simulink library "Model_DG_Grid_Following_Converter"  (R2023b)
settings: Solver=VariableStepAuto  StartTime=0.0  StopTime=10.0  RelTol=1e-3
undefined symbols (not defined in the file): K_Matching, Luenberger_Gain, ss_plant, ss_ref, Ts_Matching
settings Model: Creator=winkens  LastModifiedBy=a.och
settings SolverCC: AlgebraicLoopSolver=TrustRegion
settings OptimizationCC: ReuseModelBlockBuffer=off
settings DebuggingCC: UnconnectedInputMsg=warning  UnconnectedOutputMsg=warning  UnconnectedLineMsg=warning
settings ModelReferenceCC: EnableRefExpFcnMdlSchedulingChecks=on
settings RTWCC: DLArmComputeVersion=19.05

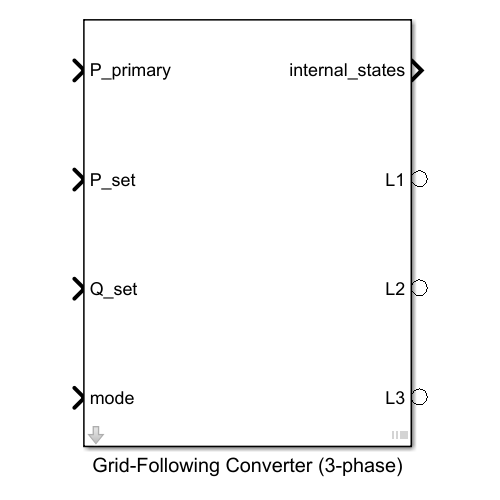
[thumbnail: Simulink's stored preview of the top-level diagram]
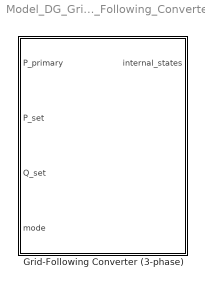
== system Model_DG_Grid_Following_Converter ==
  Grid-Following Converter (3-phase) : Subsystem  mask{S_n=30e3, P_binst=30e3, V_n_phph=400, f_n=50, send_messages=on, T_s_ctrl=1e-4, T_s_PWM_meas=1e-4, T_s_SPS=1e-4, datatype='double', swModeling=Average Model, f_sw=5e3, L_filter_conv_pu=[ 0.0001 0.05097 ], C_filter_pu=[ 0.06875 0.04569 ], L_filter_grid_pu=[ 0.01 0.04 ], withTransformer=Direct grid coupling of converter, V_n_grid_phph=20e3, RL_Trafo_Conv=[ 0.005 0.02 ], RL_Trafo_Grid=[ 0.005 0.02 ], Rm=500, Lm=500, meas_LPF=on, meas_LPF_f_cutoff=2500, prot_variant=tDMSquared warnings only, prot_v_ac_max=1.1, prot_t_ac_max=0.1, prot_v_ac_maxmax=1.25, prot_t_ac_maxmax=0.1, prot_v_ac_min=0.8, prot_t_ac_min=3, prot_v_ac_minmin=0.45, prot_t_ac_minmin=0.3, prot_f_ac_max=51.5, prot_t_f_ac_max=0.1, prot_f_ac_maxmax=52.5, prot_t_f_ac_maxmax=10, prot_f_ac_min=47.5, prot_t_f_ac_min=0.1, prot_i_ac_max=1.3, unitCtrlMode=VDE 4110, VDE4110_Pf_DBlow=49.8, VDE4110_Pf_DBhigh=50.2, VDE4110_Pf_droop=5, VDE4110_Pf_dPdt_max=1, VDE4110_Pf_T_LPF=33e-3, VDE4110_Pf_isStorage=on, ts_matching=0%Ts_Matching, k_matching=0%K_Matching, plant_ref_m=0%ss_ref, plant_model_m=0%ss_plant, luenberger_m=0%Luenberger_Gain, VDE4110_Q_Mode=(a) Q(V)-curve, VDE4110_Q_T_PT1=3.33, VDE4110_uq0ref=1, VDE4110_qmax=0.33, VDE4110_umax=1.04, VDE4110_deadband=0, VDE4110_p_pu=[0.1, 0.5, 0.6, 0.9, 1.0], VDE4110_q_pu=[0.0, 0.0, -0.05, -0.33, -0.33], VDE4110_p1=[0.94, 0.33], VDE4110_p2=[0.96, 0], VDE4110_p3=[1.04, 0], VDE4110_p4=[1.06, -0.33], VDE4110_cosphi_ref=1, VDE4110_Q_direction=Inductive Q injection, InnerCtrl_PQ_Ctrl_Mode=Closed loop, InnerCtrl_Kp_PQ=0.6, InnerCtrl_Ki_PQ=3.2, InnerCtrl_Kp=0.6, InnerCtrl_Ki=0.6, InnerCtrl_v_conv_max=1.3, InnerCtrl_i_conv_max=1.1, InnerCtrl_AD_activated=on, InnerCtrl_AD_Rvirt=0.2}
      mask prompts: S_n "Nominal Apparent Power [VA]"; P_binst "Installed Active Power [W]"; V_n_phph "Nominal Converter Voltage (rms, phase-to-phase) [V]"; f_n "Nominal Frequency [Hz]"; send_messages "Send tDMSquared info messages"; T_s_ctrl "Controller sample time [s]"; T_s_PWM_meas "PWM and measurements sample time [s]"; T_s_SPS "Simscape SPS sample time [s]"; datatype "Signal data type"; swModeling "Model type:"; f_sw "Switching Frequency [Hz]"; L_filter_conv_pu "Impedance of Converter-Side-Inductor [ R L ] (p.u.)"; C_filter_pu "Impedance of Filter Capacitor [ R C ] (p.u.)"; L_filter_grid_pu "Impedance of Grid-Side Inductor* [ R L ] (p.u.)"; V_n_grid_phph "Nominal Grid Voltage (rms, phase-to-phase) [V]"; RL_Trafo_Conv "Converter-Side Impedance [ R L ] (pu)"; RL_Trafo_Grid "Grid-Side Impedance [ R L ] (pu)"; Rm "Magnetization resistance Rm (pu)"; Lm "Magnetization inductance Lm (pu)"; meas_LPF "Apply low pass filtering to measured signals"; meas_LPF_f_cutoff "Cutoff frequency of the low pass filter applied to measurements [Hz]"; prot_variant "Protection variant"; prot_v_ac_max "Maximum AC voltage [% nom. value]"; prot_t_ac_max "Maximum AC voltage timing [s]"; prot_v_ac_maxmax "Upper Maximum AC voltage [% nom. value]"; prot_t_ac_maxmax "Upper Maximum AC voltage timing [s]"; prot_v_ac_min "Upper Minimum AC voltage [% nom. value]"; prot_t_ac_min "Upper Minimum AC voltage timing [s]"; prot_v_ac_minmin "Lower Minimum AC voltage [% nom. value]"; prot_t_ac_minmin "Lower Minimum AC voltage timing [s]"; prot_f_ac_max "Maximum AC frequency [Hz]"; prot_t_f_ac_max "Maximum AC frequency timing [s]"; prot_f_ac_maxmax "Upper Maximum AC frequency [Hz]"; prot_t_f_ac_maxmax "Upper Maximum AC frequency timing [s]"; prot_f_ac_min "Minimum AC frequency [Hz]"; prot_t_f_ac_min "Minimum AC frequency timing [s]"; prot_i_ac_max "Maximum AC current [% nom. value]"; unitCtrlMode "Unit Control Mode"; VDE4110_Pf_DBlow "P(f) Deadband Lower Limit [Hz]"; VDE4110_Pf_DBhigh "P(f) Deadband Upper Limit [Hz]"; VDE4110_Pf_droop "P(f) Droop [(df/f_n)/(dP/Pref)] [%]"; VDE4110_Pf_dPdt_max "P(f) Maximum dP/dt [pu / s]"; VDE4110_Pf_T_LPF "P(f) time constant of active power PT1 delay [s]"; VDE4110_Pf_isStorage "Generation Unit Is Energy Storage"; ts_matching "Time Constant"; k_matching "Feedback Gain"; plant_ref_m "Reference Model"; plant_model_m "Plant Model"; luenberger_m "Luenberger Gain"; VDE4110_Q_Mode "Q-Control Mode"; VDE4110_Q_T_PT1 "Time constant of reactive power PT1 delay [s]"; VDE4110_uq0ref "U_Q0ref [pu]"; VDE4110_qmax "|Q_max| [pu]"; VDE4110_umax "U_max [pu]"; VDE4110_deadband "Voltage Deadband [+- %]"; VDE4110_p_pu "P_grid points [pu]"; VDE4110_q_pu "Q_grid points [pu]"; VDE4110_p1 "P1 [V_grid, Q_grid] [pu]"; VDE4110_p2 "P2 [V_grid, Q_grid] [pu]"; VDE4110_p3 "P3 [V_grid, Q_grid] [pu]"; VDE4110_p4 "P4 [V_grid, Q_grid] [pu]"; VDE4110_cosphi_ref "cos(phi)"; InnerCtrl_PQ_Ctrl_Mode "Control mode"; InnerCtrl_Kp_PQ "Power controller proportional gain [p.u.]"; InnerCtrl_Ki_PQ "Power controller integral gain [p.u.]"; InnerCtrl_Kp "Current Controller Proportional Gain [p.u.]"; InnerCtrl_Ki "Current Controller Integral Gain [p.u.]"; InnerCtrl_v_conv_max "Converter voltage maximum value (limit) [p.u.]"; InnerCtrl_i_conv_max "Converter current maximum value (limit) [p.u.]"; InnerCtrl_AD_activated "Active damping activated"; InnerCtrl_AD_Rvirt "Virtual resistor for active damping (in series with conv.-side inductance) [p.u.]"
      mask init:
      | % Initialize nominal grid voltage
      | if (withTransformer == 1)
      |     V_n_grid_phph = V_n_phph;
      | end
      mask TypeOptions swModeling: Average Model | Ideal Switches
      mask TypeOptions withTransformer: Direct grid coupling of converter | Grid coupling using transformer
      mask Callback withTransformer:
      | msk = Simulink.Mask.get(gcb);
      | p = msk.Parameters;
      | if strcmp(get_param(gcb, 'withTransformer'), 'Grid coupling using transformer')
      |     %with Transformer
      |     p(16).Visible = 'on';
      |     p(17).Visible = 'on';
      |     p(18).Visible = 'on';
      |     p(19).Visible = 'on';
      |     p(20).Visible = 'on';
      | else
      |     %without Transformer
      |     p(16).Visible = 'off';
      |     p(17).Visible = 'off';
      |     p(18).Visible = 'off';
      |     p(19).Visible = 'off';
      |     p(20).Visible = 'off';
      | end
      mask TypeOptions prot_variant: Hardware protection | tDMSquared warnings only | deactivated | VDE AR
      mask Callback prot_variant:
      | msk = Simulink.Mask.get(gcb);
      | if strcmp(get_param(gcb, 'prot_variant'), 'VDE AR')
      |     msk.getParameter('prot_v_ac_max').Visible ='on';
      |     msk.getParameter('prot_i_ac_max').Visible ='on';
      |     msk.getParameter('prot_t_ac_max').Visible = 'on';
      |     msk.getParameter('prot_v_ac_maxmax').Visible = 'on';
      |     msk.getParameter('prot_t_ac_maxmax').Visible = 'on';
      |     msk.getParameter('prot_v_ac_min').Visible = 'on';
      |     msk.getParameter('prot_t_ac_min').Visible = 'on';
      |     msk.getParameter('prot_v_ac_minmin').Visible = 'on';
      |     msk.getParameter('prot_t_ac_minmin').Visible = 'on';
      |     msk.getParameter('prot_f_ac_max').Visible = 'on';
      |     msk.getParameter('prot_t_f_ac_max').Visible = 'on';
      |     msk.getParameter('prot_f_ac_maxmax').Visible = 'on';
      |     msk.getParameter('prot_t_f_ac_maxmax').Visible = 'on';
      |     msk.getParameter('prot_f_ac_min').Visible = 'on';
      |     msk.getParameter('prot_t_f_ac_min').Visible = 'on';
      | elseif strcmp(get_param(gcb, 'prot_variant'), 'deactivated')
      |     msk.getParameter('prot_v_ac_max').Visible ='off';
      |     msk.getParameter('prot_i_ac_max').Visible ='off';
      |     msk.getParameter('prot_t_ac_max').Visible = 'off';
      |     msk.getParameter('prot_v_ac_maxmax').Visible = 'off';
      |     msk.getParameter('prot_t_ac_maxmax').Visible = 'off';
      |     msk.getParameter('prot_v_ac_min').Visible = 'off';
      |     msk.getParameter('prot_t_ac_min').Visible = 'off';
      |     msk.getParameter('prot_v_ac_minmin').Visible = 'off';
      |     msk.getParameter('prot_t_ac_minmin').Visible = 'off';
      |     msk.getParameter('prot_f_ac_max').Visible = 'off';
      |     msk.getParameter('prot_t_f_ac_max').Visible = 'off';
      |     msk.getParameter('prot_f_ac_maxmax').Visible = 'off';
      |     msk.getParameter('prot_t_f_ac_maxmax').Visible = 'off';
      |     msk.getParameter('prot_f_ac_min').Visible = 'off';
      |     msk.getParameter('prot_t_f_ac_min').Visible = 'off';
      | else
      |     msk.getParameter('prot_v_ac_max').Visible ='on';
      |     msk.getParameter('prot_i_ac_max').Visible ='on';
      |     msk.getParameter('prot_t_ac_max').Visible = 'off';
      |     msk.getParameter('prot_v_ac_maxmax').Visible = 'off';
      |     msk.getParameter('prot_t_ac_maxmax').Visible = 'off';
      |     msk.getParameter('prot_v_ac_min').Visible = 'off';
      |     msk.getParameter('prot_t_ac_min').Visible = 'off';
      |     msk.getParameter('prot_v_ac_minmin').Visible = 'off';
      |     msk.getParameter('prot_t_ac_minmin').Visible = 'off';
      |     msk.getParameter('prot_f_ac_max').Visible = 'off';
      |     msk.getParameter('prot_t_f_ac_max').Visible = 'off';
      |     msk.getParameter('prot_f_ac_maxmax').Visible = 'off';
      |     msk.getParameter('prot_t_f_ac_maxmax').Visible = 'off';
      |     msk.getParameter('prot_f_ac_min').Visible = 'off';
      |     msk.getParameter('prot_t_f_ac_min').Visible = 'off';
      | end
      mask TypeOptions unitCtrlMode: VDE 4110 | Matching Control | No Unit Control
      mask Callback unitCtrlMode:
      | toggleComment = @(s) regexprep( ...
      |     regexprep(s,'^$','0'), ...       % leere Eingabe → '0'
      |     '^(?!0%)(.*)', ...               % Negative Lookahead: wenn nicht '0%' am Anfang
      |     '0%$1' ...                       % dann '0%' voranstellen
      | );
      | 
      | removeComment = @(s) regexprep( ...
      |     regexprep(s,'^$','0'), ...       % leere Eingabe → '0'
      |     '^0%', ...                       % wenn '0%' am Anfang steht
      |     '' ...                           % entferne es
      | );
      |     m = Simulink.Mask.get(gcb);
      | 
      |     modeStr = get_param(gcb, 'unitCtrlMode');
      | 
      |     % 3) Liste der zu „auskommentierenden“ Controls je Modus
      |     vdeControls      = {'VDE4110_Pf_dPdt_max', 'VDE4110_Pf_DBlow', 'VDE4110_Pf_DBhigh', 'VDE4110_Pf_droop', 'VDE4110_Pf_T_LPF'};
      |     matchingControls = {'ts_matching', 'k_matching', 'plant_ref_m', 'plant_model_m', 'luenberger_m'};
      | 
      |     switch modeStr
      |         case 'VDE 4110'
      |             m.getDialogControl('paramboxVDE4110').Visible = 'on';
      |             m.getDialogControl('paramboxMatching').Visible = 'off';
      |             m.getDialogControl('paramboxReactiveCtrl').Visible = 'on';
      |             % → Matching-Felder a u s k o m m e n t i e r e n
      |             for i = 1:numel(matchingControls)
      |                 set_param(gcb, matchingControls{i}, (toggleComment(get_param(gcb, matchingControls{i}))));
      |             end
      |             % → VDE-Felder e n t k o m m e n t i e r e n
      |             for i = 1:numel(vdeControls)
      |                 set_param(gcb, vdeControls{i}, (removeComment(get_param(gcb, vdeControls{i}))));
      |             end
      | 
      |         case 'Matching Control'
      |             m.getDialogControl('paramboxVDE4110').Visible = 'off';
      |             m.getDialogControl('paramboxMatching').Visible = 'on';
      |             m.getDialogControl('paramboxReactiveCtrl').Visible = 'on';
      |             % → VDE-Felder a u s k o m m e n t i e r e n
      |             for i = 1:numel(vdeControls)
      |                 set_param(gcb, vdeControls{i}, (toggleComment(get_param(gcb, vdeControls{i}))));
      |             end
      |             % → Matching-Felder e n t k o m m e n t i e r e n
      |             for i = 1:numel(matchingControls)
      |                 set_param(gcb, matchingControls{i}, (removeComment(get_param(gcb, matchingControls{i}))));
      |             end
      |         case 'No Unit Control'
      |             m.getDialogControl('paramboxVDE4110').Visible = 'off';
      |             m.getDialogControl('paramboxMatching').Visible = 'off';
      |             m.getDialogControl('paramboxReactiveCtrl').Visible = 'off';
      |             % → VDE-Felder a u s k o m m e n t i e r e n
      |             for i = 1:numel(vdeControls)
      |                 set_param(gcb, vdeControls{i}, (toggleComment(get_param(gcb, vdeControls{i}))));
      |             end
      |             % → Matching-Felder e n t k o m m e n t i e r e n
      |             for i = 1:numel(matchingControls)
      |                 set_param(gcb, matchingControls{i}, (toggleComment(get_param(gcb, matchingControls{i}))));
      |             end
      |     end
      mask TypeOptions VDE4110_Q_Mode: (a) Q(V)-curve | (b) Q(P)-curve | (c) Constant Q with Q(V)-limitation | (d) Constant cos(phi)
      mask Callback VDE4110_Q_Mode:
      | msk = Simulink.Mask.get(gcb);
      | p = msk.Parameters;
      | if strcmp(get_param(gcb, 'VDE4110_Q_Mode'), '(a) Q(V)-curve')
      |     %(a) Q(V)
      |     msk.getDialogControl('paramboxVDE4110_Q_a').Visible = 'on';
      |     msk.getDialogControl('paramboxVDE4110_Q_b').Visible = 'off';
      |     msk.getDialogControl('paramboxVDE4110_Q_c').Visible = 'off';
      |     msk.getDialogControl('paramboxVDE4110_Q_d').Visible = 'off';
      | elseif strcmp(get_param(gcb, 'VDE4110_Q_Mode'), '(b) Q(P)-curve')
      |     %(b) Q(P)
      |     msk.getDialogControl('paramboxVDE4110_Q_a').Visible = 'off';
      |     msk.getDialogControl('paramboxVDE4110_Q_b').Visible = 'on';
      |     msk.getDialogControl('paramboxVDE4110_Q_c').Visible = 'off';
      |     msk.getDialogControl('paramboxVDE4110_Q_d').Visible = 'off';
      | elseif strcmp(get_param(gcb, 'VDE4110_Q_Mode'), '(c) Constant Q with Q(V)-limitation')
      |     %(c) const Q
      |     msk.getDialogControl('paramboxVDE4110_Q_a').Visible = 'off';
      |     msk.getDialogControl('paramboxVDE4110_Q_b').Visible = 'off';
      |     msk.getDialogControl('paramboxVDE4110_Q_c').Visible = 'on';
      |     msk.getDialogControl('paramboxVDE4110_Q_d').Visible = 'off';
      | else
      |     %(d) const cosphi
      |     msk.getDialogControl('paramboxVDE4110_Q_a').Visible = 'off';
      |     msk.getDialogControl('paramboxVDE4110_Q_b').Visible = 'off';
      |     msk.getDialogControl('paramboxVDE4110_Q_c').Visible = 'off';
      |     msk.getDialogControl('paramboxVDE4110_Q_d').Visible = 'on';
      | end
      mask TypeOptions VDE4110_Q_direction: Inductive Q injection | Inductive Q consumption
      mask TypeOptions InnerCtrl_PQ_Ctrl_Mode: Closed loop | Open loop
      mask DialogControl title Prompt: Grid-Following Converter (3-phase)
      mask DialogControl modelDescription Prompt: Three-phase converter model representing distributed generation units. Power electronics can either be modeled as switches or as average model.
      mask DialogControl tabGeneral Prompt: General
      mask DialogControl paramboxSamplesData Prompt: Sample Times and Data Types
      mask DialogControl tabElectrical Prompt: Electrical Part
      mask DialogControl containerSwitches Prompt: Modeling of Switches
      mask DialogControl paramboxLCL Prompt: Filter and DC components
      mask DialogControl textLCL Prompt: The filter parameters are defined in a per-unit-system based on the nominal power, the nominal frequency and the nominal converter-side voltage defined in tab General.
      mask DialogControl Control6 Prompt: *Only if no transformer is used.
      mask DialogControl paramboxTrafo Prompt: Transformer Parameters
      mask DialogControl textTrafo Prompt: Transformer parameters are defined in a per-unit-system based on the nominal power, the nominal frequency and the nominal voltages defined here and in tab General. The reference voltage for the impedance values depends on the respective nominal voltage level. However, magnetization resistance and inductance are based on the generator-side nominal voltage.
      mask DialogControl Container22 Prompt: Measurements
      mask DialogControl Control7 Prompt: These parameters are related to the processing of the measurement signals.
      mask DialogControl Container25 Prompt: Protection parameters
      mask DialogControl tabUnitCtrl Prompt: Unit Control
      mask DialogControl paramboxActiveCtrl Prompt: Active Power Control
      mask DialogControl paramboxVDE4110 Prompt: VDE 4110 Parameters
      mask DialogControl paramboxMatching Prompt: Matching Control Models
      mask DialogControl paramboxReactiveCtrl Prompt: Reactive Power Control
      mask DialogControl paramboxVDE4110_Q_a Prompt: Q(V) Parameters
      mask DialogControl paramboxVDE4110_Q_b Prompt: Q(P) Parameters
      mask DialogControl paramboxVDE4110_Q_c Prompt: Constant Q with Q(V)-Limitation Parameters
      mask DialogControl paramboxVDE4110_Q_d Prompt: Constant cos(phi) Parameters
      mask DialogControl tabInnerCtrl Prompt: Inner Control
      mask DialogControl textInnerControl Prompt: The inner control parameters are given in per-unit. The reference voltage and current are the amplitude of the nominal phase-to-neutral voltage and the amplitude of the phase current, respectively. The reference power is the converter apparent power.
      mask DialogControl paramboxPQCtrl Prompt: Active and reactive power controller
      mask DialogControl paramboxInnerCtrl Prompt: PI current controller
      mask DialogControl Container30 Prompt: Active damping

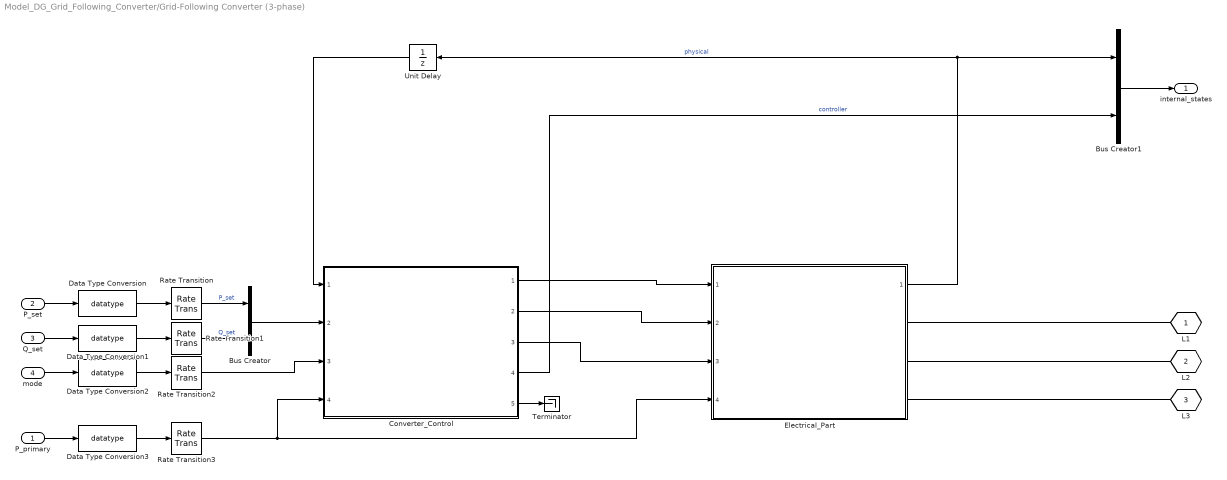
== system Model_DG_Grid_Following_Converter/Grid-Following Converter (3-phase) ==
  P_primary : Inport
  P_set : Inport  Port=2
  Q_set : Inport  Port=3
  mode : Inport  Port=4
  Bus Creator : BusCreator  Inputs=2
  Bus Creator1 : BusCreator  Inputs=2
  Converter_Control : Subsystem  ReferencedSubsystem=Subsys_GFolConv_Control  S_n=S_n  P_binst=P_binst  f_n=f_n  V_n_phph=V_n_phph  V_n_grid_phph=V_n_grid_phph  V_n_dc=2*V_n_phph  L_filter_conv_pu=L_filter_conv_pu  C_filter_pu=C_filter_pu  outputSignal=swModeling - 1  f_sw=f_sw  send_info_messages=send_messages  T_s_ctrl=T_s_ctrl  T_s_PWM_meas=T_s_PWM_meas  datatype=datatype  meas_signals=0  meas_lowpass=meas_LPF  meas_f_cutoff_lowpass=meas_LPF_f_cutoff  meas_f_cutoff_posseq=20  prot_variant=prot_variant  v_dc_max=1.2  v_ac_max=prot_v_ac_max  t_ac_max=prot_t_ac_max  v_ac_maxmax=prot_v_ac_maxmax  t_ac_maxmax=prot_t_ac_maxmax  v_ac_min=prot_v_ac_min  t_ac_min=prot_t_ac_min  v_ac_minmin=prot_v_ac_minmin  t_ac_minmin=prot_t_ac_minmin  f_ac_max=prot_f_ac_max  t_f_ac_max=prot_t_f_ac_max  f_ac_maxmax=prot_f_ac_maxmax  t_f_ac_maxmax=prot_t_f_ac_maxmax  f_ac_min=prot_f_ac_min  t_f_ac_min=prot_t_f_ac_min  i_ac_max=prot_i_ac_max  outer_ctrl_mode=unitCtrlMode  VDE4110_T_LPF_P=VDE4110_Pf_T_LPF  VDE4110_Pf_DBlow=VDE4110_Pf_DBlow  VDE4110_Pf_DBhigh=VDE4110_Pf_DBhigh  VDE4110_Pf_droop=VDE4110_Pf_droop  VDE4110_Pf_dPdtmax=VDE4110_Pf_dPdt_max  isStorage=VDE4110_Pf_isStorage  Ts_Matching_m=ts_matching  K_Matching_m=k_matching  Plant_Ref=plant_ref_m  Plant_Model=plant_model_m  Luenberger=luenberger_m  VDE4110_Q_ctrl_mode=VDE4110_Q_Mode  VDE4110_T_PT1_Q=VDE4110_Q_T_PT1  VDE4110_QV_uq0ref=VDE4110_uq0ref  VDE4110_QV_qmax=VDE4110_qmax  VDE4110_QV_umax=VDE4110_umax  VDE4110_QV_deadband=VDE4110_deadband  VDE4110_QP_P=VDE4110_p_pu  VDE4110_QP_Q=VDE4110_q_pu  VDE4110_QVDB_P1=VDE4110_p1  VDE4110_QVDB_P2=VDE4110_p2  VDE4110_QVDB_P3=VDE4110_p3  VDE4110_QVDB_P4=VDE4110_p4  VDE4110_cosphi_ref=VDE4110_cosphi_ref  VDE4110_cosphi_direction=2 - VDE4110_Q_direction  PQ_ctrl_mode=InnerCtrl_PQ_Ctrl_Mode - 1  K_p_PQ_Ctrl=InnerCtrl_Kp_PQ  K_i_PQ_Ctrl=InnerCtrl_Ki_PQ  K_p_I_Ctrl=InnerCtrl_Kp  K_i_I_Ctrl=InnerCtrl_Ki  v_conv_max=InnerCtrl_v_conv_max  i_grid_max=InnerCtrl_i_conv_max  active_damping=InnerCtrl_AD_activated  R_virt_pu=InnerCtrl_AD_Rvirt
  Data Type Conversion{,1..3} (4 alike) : DataTypeConversion  OutDataTypeStr=datatype  SaturateOnIntegerOverflow=off  RndMeth=Floor
  Electrical_Part : Subsystem  ReferencedSubsystem=Subsys_Conv_Electrical_Part_SPS  S_n=S_n  f_n=f_n  V_n_phph=V_n_phph  V_n_grid_phph=V_n_grid_phph  T_s_ctrl=T_s_ctrl  T_s_meas=T_s_PWM_meas  T_s_SPS=T_s_SPS  datatype=datatype  L_filter_conv_pu=L_filter_conv_pu  C_filter_pu=C_filter_pu  L_filter_grid_pu=L_filter_grid_pu  withTransformer=withTransformer - 1  RL_Trafo_Conv=RL_Trafo_Conv  RL_Trafo_Grid=RL_Trafo_Grid  Rm=Rm  Lm=Lm  inverterModel=2 - swModeling  R_snubber_pu=5e6  R_on_pu=1e-3  energySourceModel=0  C_dc_pu=0.75  K_p_DC=1.2  K_i_DC=2.4
  Rate Transition{,1..3} (4 alike) : RateTransition  OutPortSampleTime=T_s_ctrl
  Terminator : Terminator
  Unit Delay : UnitDelay  SampleTime=-1  HasFrameUpgradeWarning=on
  L1 : PMIOPort  Tag=PMCPort  Side=Right
  L2 : PMIOPort  Tag=PMCPort  Port=2  Side=Right
  L3 : PMIOPort  Tag=PMCPort  Port=3  Side=Right
  internal_states : Outport
  wires:
  Bus Creator1/1 -> internal_states/1
  P_primary/1 -> Data Type Conversion3/1
  P_set/1 -> Data Type Conversion/1
  Q_set/1 -> Data Type Conversion1/1
  Electrical_Part/1 -> Bus Creator1/1, Unit Delay/1  "physical"
  Converter_Control/1 -> Electrical_Part/1
  Converter_Control/2 -> Electrical_Part/2
  Converter_Control/3 -> Electrical_Part/3
  Converter_Control/5 -> Terminator/1
  Converter_Control/4 -> Bus Creator1/2  "controller"
  Unit Delay/1 -> Converter_Control/1
  Bus Creator/1 -> Converter_Control/2
  mode/1 -> Data Type Conversion2/1
  Data Type Conversion/1 -> Rate Transition/1
  Data Type Conversion1/1 -> Rate Transition1/1
  Data Type Conversion2/1 -> Rate Transition2/1
  Data Type Conversion3/1 -> Rate Transition3/1
  Rate Transition/1 -> Bus Creator/1  "P_set"
  Rate Transition1/1 -> Bus Creator/2  "Q_set"
  Rate Transition2/1 -> Converter_Control/3
  Rate Transition3/1 -> Converter_Control/4, Electrical_Part/4
  connections:
  Electrical_Part/RConn1 -- L1/RConn1
  Electrical_Part/RConn2 -- L2/RConn1
  Electrical_Part/RConn3 -- L3/RConn1
